simulink model "control"  (R2024a)
settings: Solver=FixedStepAuto  StartTime=0.0  StopTime=48  FixedStep=0.001  RelTol=1e-3  EnableMultiTasking=on
undefined symbols (not defined in the file): C_b, Cdr_off, M_b, M_off
settings Model: Creator=simil  LastModifiedBy=simil
settings SolverCC: AutoInsertRateTranBlk=on
settings OptimizationCC: UseDivisionForNetSlopeComputation=on
settings DebuggingCC: MultiTaskCondExecSysMsg=none  MultiTaskRateTransMsg=warning

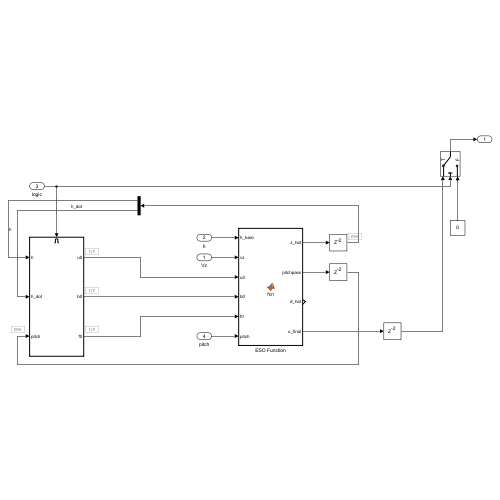
[thumbnail: Simulink's stored preview of the top-level diagram]
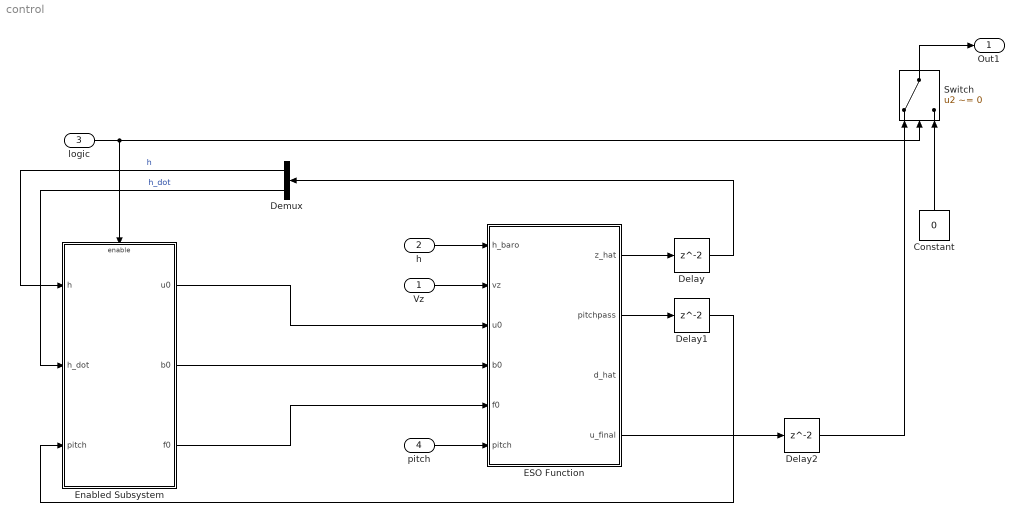
== system control ==
  Vz : Inport
  h : Inport  Port=2
  logic : Inport  Port=3  OutDataTypeStr=boolean
  pitch : Inport  Port=4
  Constant : Constant  Value=0
  Delay : Delay
  Delay1 : Delay
  Delay2 : Delay
  Demux : Demux  Outputs=2
  ESO Function : MATLAB Function  TreatAsAtomicUnit=on  SystemSampleTime=0.001
  Enabled Subsystem : Subsystem  TreatAsAtomicUnit=on
  Switch : Switch  Criteria=u2 ~= 0  SaturateOnIntegerOverflow=off  InputSameDT=off
  Out1 : Outport
  wires:
  ESO Function/4(u_final) -> Delay2/1
  Demux/2 -> Enabled Subsystem/2(h_dot)  "h_dot"
  Demux/1 -> Enabled Subsystem/1(h)  "h"
  Delay2/1 -> Switch/1
  Constant/1 -> Switch/3
  Enabled Subsystem/3(f0) -> ESO Function/5(f0)
  ESO Function/2(pitchpass) -> Delay1/1
  Delay1/1 -> Enabled Subsystem/3(pitch)
  ESO Function/1(z_hat) -> Delay/1
  Enabled Subsystem/1(u0) -> ESO Function/3(u0)
  Enabled Subsystem/2(b0) -> ESO Function/4(b0)
  logic/1 -> Enabled Subsystem/Enable, Switch/2
  Switch/1 -> Out1/1
  Vz/1 -> ESO Function/2(vz)
  Delay/1 -> Demux/1
  h/1 -> ESO Function/1(h_baro)
  pitch/1 -> ESO Function/6(pitch)

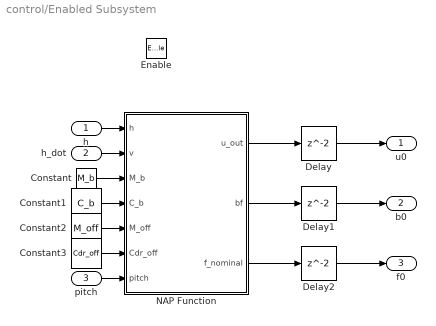
== system control/Enabled Subsystem ==
  h : Inport
  h_dot : Inport  Port=2
  pitch : Inport  Port=3
  Enable : EnablePort
  Constant : Constant  Value=M_b
  Constant1 : Constant  Value=C_b
  Constant2 : Constant  Value=M_off
  Constant3 : Constant  Value=Cdr_off
  Delay : Delay
  Delay1 : Delay
  Delay2 : Delay
  NAP Function : MATLAB Function  TreatAsAtomicUnit=on  SystemSampleTime=0.01
  u0 : Outport
  b0 : Outport  Port=2
  f0 : Outport  Port=3
  wires:
  Constant/1 -> NAP Function/3(M_b)
  Constant2/1 -> NAP Function/5(M_off)
  Constant3/1 -> NAP Function/6(Cdr_off)
  Constant1/1 -> NAP Function/4(C_b)
  h/1 -> NAP Function/1(h)
  h_dot/1 -> NAP Function/2(v)
  pitch/1 -> NAP Function/7(pitch)
  NAP Function/1(u_out) -> Delay/1
  NAP Function/2(bf) -> Delay1/1
  NAP Function/3(f_nominal) -> Delay2/1
  Delay/1 -> u0/1
  Delay1/1 -> b0/1
  Delay2/1 -> f0/1

== matlab function control/ESO Function ==
  data: h_baro input; z_hat output; pitchpass output; vz input; u0 input; b0 input; f0 input; pitch input; d_hat output; u_final output
function [z_hat,pitchpass,d_hat, u_final] = fcn(h_baro, vz, u0, b0, f0, pitch)
%#codegen
omega = 6;
if isnan(u0), u0 = 0; end
if isnan(b0) || b0 == 0, b0 = -5; end
if isnan(f0), f0 = -9.81; end
pitchpass = pitch;

persistent z1 z2 z3 u_prev
stepsize = 0.001;
if isempty(z1)
    z1 = 892; z2 = 0; z3 = -9.81; u_prev = 0;
    if ~isnan(h_baro), z1 = h_baro; end
    if ~isnan(vz), z2 = vz; end
    if ~isnan(f0), z3 = f0; end
end

if isnan(h_baro) || isnan(vz)
    z_hat = [z1; z2];
    d_hat = z3;
    u_final = u_prev;
else
    beta1 = 3 * omega;
    beta2 = 3 * (omega^2);
    beta3 = omega^3;
    e = z1 - h_baro;
    max_rate = 0.3;
    delta_correction = max(-0.5, min(0.5, -z3 / b0));
    u_raw = u0 + delta_correction;
    u_ratelimited = u_prev + max(min(u_raw - u_prev, max_rate), -max_rate);
    u_final = max(0.0, min(1.0, u_ratelimited));

    z1_next = z1 + stepsize*(z2 - beta1*e);
    z2_next = z2 + stepsize*(z3 + f0 - beta2*e + b0*u_final);
    z3_next = z3 + stepsize*(-beta3*e);
    z1 = z1_next;
    z2 = z2_next;
    z3 = z3_next;
    u_prev = u_final;
    z_hat = [z1; z2];
    d_hat = z3;
end
end

== matlab function control/Enabled Subsystem/NAP Function ==
  settings: updateMethod=DISCRETE
  data: h input; u_out output; v input; M_b input; C_b input; M_off input; Cdr_off input; pitch input; bf output; f_nominal output
function [u_out,bf,f_nominal] = NAP(h,v,M_b,C_b,M_off,Cdr_off,pitch)
    u_out = 0; 
    bf = -4.5;
    f_nominal = -9.81;
    persistent tick u_store bf_store f_store

    if isempty(tick)
        tick = 0;    
        u_store = 0;
        bf_store = bf;
        f_store = f_nominal;
    end

    if isnan(h) || isnan(v)
       return
    end

if tick <= 0
    h_target = (33400)*0.3048+892;
    [h_pred_min,bf_min,f_min] = RK2(h, v, pitch, 0.0, M_b, C_b, M_off, Cdr_off);
    
    if h_pred_min < h_target
        u_out = 0.0;
        bf = bf_min;
        f_nominal = f_min;
        return;
    end
    [h_pred_max,bf_max,f_max] = RK2(h, v, pitch, 1.0, M_b, C_b, M_off, Cdr_off);
    if h_pred_max > h_target
        u_out = 1.0;
        bf = bf_max;
        f_nominal = f_max;
        return;
    end

    u_low = 0.0;
    u_high = 1.0;
    u_mid = 0.5;

    for iter = 1:5
        [h_sim,current_bf,current_f] = RK2(h, v, pitch, u_mid, M_b, C_b, M_off, Cdr_off);
        bf_store = current_bf;
        f_store = current_f;
        if h_sim > h_target
            u_low = u_mid;
        else
            u_high = u_mid;
        end
        u_mid = (u_low + u_high) / 2;
    end
    u_out = u_mid; 
    u_store = u_out;
    tick = 10;
end
    tick = tick - 1;
    u_out = u_store;
    bf = bf_store;
    f_nominal = f_store;
end

function [h_final,bf,f] = RK2(h, v, pitch, u_val, M_b, C_b, M_off, Cdr_off)
    m = 25.142; Ar = pi*(0.131/2)^2; Ab = 2*1111.162e-6; g = 9.81;         
    dt = 0.1;      
    h1 = h;
    v1 = v;
    stream0 = v / cos(pitch);
    T0 = 288.15 - 0.0065 * h;
    P0 = 101325 * (T0 / 288.15)^5.2558;
    rho0 = P0 / (287.0528 * T0);
    mach0 = stream0/sqrt(1.4*287.0528*T0);
    Cdb0 = interp1(M_b, C_b, mach0, 'linear', 'extrap');
    Cdr0 = interp1(M_off, Cdr_off, mach0, 'linear', 'extrap');
    bf = (-0.5 * rho0 * stream0^2 * Cdb0 * Ab / m) * cos(pitch);
    f = (-0.5 * rho0 * stream0^2 * Cdr0 * Ar / m) * cos(pitch) - g;
   
    max_iter = 500;
    for iter_rk = 1:max_iter
        if v1 < 0, break; end
        stream1 = v1/cos(pitch);
        T1 = 288.15 - 0.0065 * h1;
        P1 = 101325 * (T1 / 288.15)^5.2558;
        rho1 = P1 / (287.0528 * T1);
        mach1 = stream1 / sqrt(1.4 * 287.0528 * T1);
        Cdb1 = interp1(M_b, C_b, mach1, 'linear', 'extrap');
        Cdr1 = interp1(M_off, Cdr_off, mach1, 'linear', 'extrap');
        b0_1 = (-0.5 * rho1 * stream1^2 * Cdb1 * Ab / m) * cos(pitch);
        f1 = (-0.5 * rho1 * stream1^2 * Cdr1 * Ar / m) * cos(pitch) - g;
        a1 = f1 + b0_1 * u_val; 
        h2 = h1 + v1 * (dt / 2);
        v2 = v1 + a1 * (dt / 2);
        stream2 = v2/cos(pitch);
        T2 = 288.15 - 0.0065 * h2;
        P2 = 101325 * (T2 / 288.15)^5.2558;
        rho2 = P2 / (287.0528 * T2);
        mach2 = stream2 / sqrt(1.4 * 287.0528 * T2);
        Cdb2 = interp1(M_b, C_b, mach2, 'linear', 'extrap');
        Cdr2 = interp1(M_off, Cdr_off, mach2, 'linear', 'extrap');
        b0_2 = (-0.5 * rho2 * stream2^2 * Cdb2 * Ab / m) * cos(pitch);
        f2 = (-0.5 * rho2 * stream2^2 * Cdr2 * Ar / m) * cos(pitch) - g;
        a2 = f2 + b0_2 * u_val; 
        v1 = v1 + a2 * dt;
        h1 = h1 + v2 * dt;
        if h1 > 12000, break; end
    end
    h_final = h1;
end
